simulink subsystem "Zone_Threshold"  (R2023b)
settings: Solver=VariableStepAuto  StartTime=0.0  StopTime=10.0  RelTol=1e-3
model mask{Max_X=0, Min_X=0, Max_Y=0, Min_Y=0, Zone_Time=0}
  mask prompts: Max_X "X Max of Threshold (meters for all)"; Min_X "X Min"; Max_Y "Y Max"; Min_Y "Y Min"
settings Model: Creator=Bing  LastModifiedBy=FIRSTMentor

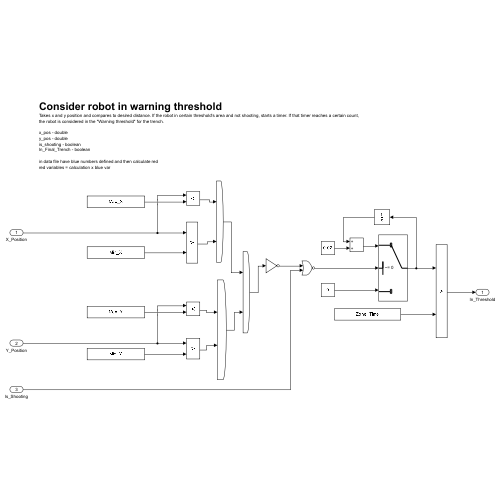
[thumbnail: Simulink's stored preview of the top-level diagram]
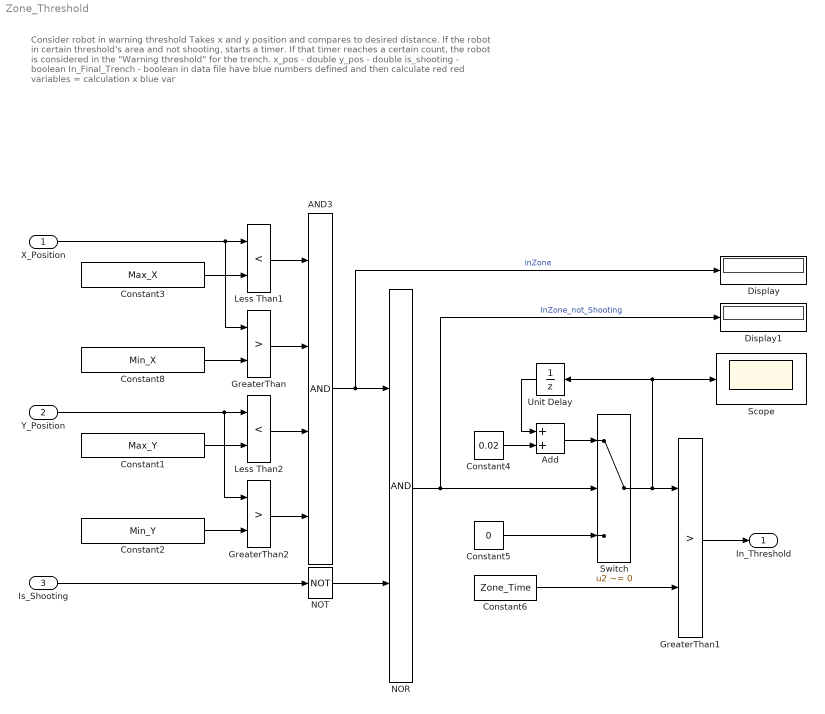
== system Zone_Threshold ==
  note: Consider robot in warning threshold
      | Takes x and y position and compares to desired distance. If the robot in certain threshold's area and not shooting, starts a timer. If that timer reaches a certain count, the robot is considered in the "Warning threshold" for the trench.
      |
      | x_pos - double
      | y_pos - double
      | is_shooting - boolean
      | In_Final_Trench - boolean
      |
      | in data file have blue numbers defined and then calculate red
      | red variables = calculation x blue var
  X_Position : Inport
  Y_Position : Inport  Port=2
  Is_Shooting : Inport  Port=3
  AND3 : Logic  Inputs=4  AllPortsSameDT=off  OutDataTypeStr=boolean
  Add : Sum
  Constant1 : Constant  Value=Max_Y
  Constant2 : Constant  Value=Min_Y
  Constant3 : Constant  Value=Max_X
  Constant4 : Constant  Value=0.02
  Constant5 : Constant  Value=0
  Constant6 : Constant  Value=Zone_Time
  Constant8 : Constant  Value=Min_X
  Display : Display
  Display1 : Display
  GreaterThan : RelationalOperator  Operator=>  OutDataTypeStr=boolean  RndMeth=Simplest  InputSameDT=off
  GreaterThan1 : RelationalOperator  Operator=>  OutDataTypeStr=boolean  RndMeth=Simplest  InputSameDT=off
  GreaterThan2 : RelationalOperator  Operator=>  OutDataTypeStr=boolean  RndMeth=Simplest  InputSameDT=off
  Less Than1 : RelationalOperator  Operator=<  OutDataTypeStr=boolean  RndMeth=Simplest  InputSameDT=off
  Less Than2 : RelationalOperator  Operator=<  OutDataTypeStr=boolean  RndMeth=Simplest  InputSameDT=off
  NOR : Logic  AllPortsSameDT=off  OutDataTypeStr=boolean
  NOT : Logic  Operator=NOT  AllPortsSameDT=off  OutDataTypeStr=boolean
  Scope : Scope
  Switch : Switch  Criteria=u2 ~= 0  SaturateOnIntegerOverflow=off  InputSameDT=off
  Unit Delay : UnitDelay  SampleTime=-1  HasFrameUpgradeWarning=on
  In_Threshold : Outport
  wires:
  Less Than1/1 -> AND3/1
  X_Position/1 -> Less Than1/1, GreaterThan/1
  Switch/1 -> Unit Delay/1, Scope/1, GreaterThan1/1
  Unit Delay/1 -> Add/1
  NOR/1 -> Display1/1, Switch/2  "InZone_not_Shooting"
  Add/1 -> Switch/1
  Constant6/1 -> GreaterThan1/2
  Constant4/1 -> Add/2
  Constant5/1 -> Switch/3
  GreaterThan1/1 -> In_Threshold/1
  Y_Position/1 -> Less Than2/1, GreaterThan2/1
  GreaterThan2/1 -> AND3/4
  AND3/1 -> Display/1, NOR/1  "inZone"
  Constant3/1 -> Less Than1/2
  Constant8/1 -> GreaterThan/2
  Constant1/1 -> Less Than2/2
  Constant2/1 -> GreaterThan2/2
  Is_Shooting/1 -> NOT/1
  GreaterThan/1 -> AND3/2
  Less Than2/1 -> AND3/3
  NOT/1 -> NOR/2
